simulink model "sonobe2025_explorer"  (R2025b)
settings: Solver=ode45  StartTime=0.0  StopTime=40  MaxStep=0.005  RelTol=1e-3
model workspace (MAT data in the model file):
  A = 62.8888888889
  Jb = 8
  Kd = 3.97
  Kp = 10.53
  Tv = 1
  g = 9.80665
  gamma = 0.02
  lb = 0.9
  mb = 60
  td = 0.155
settings Model: Creator=seguchi  LastModifiedBy=seguchi

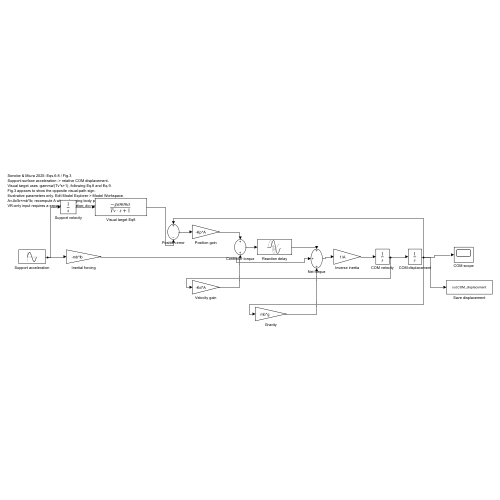
[thumbnail: Simulink's stored preview of the top-level diagram]
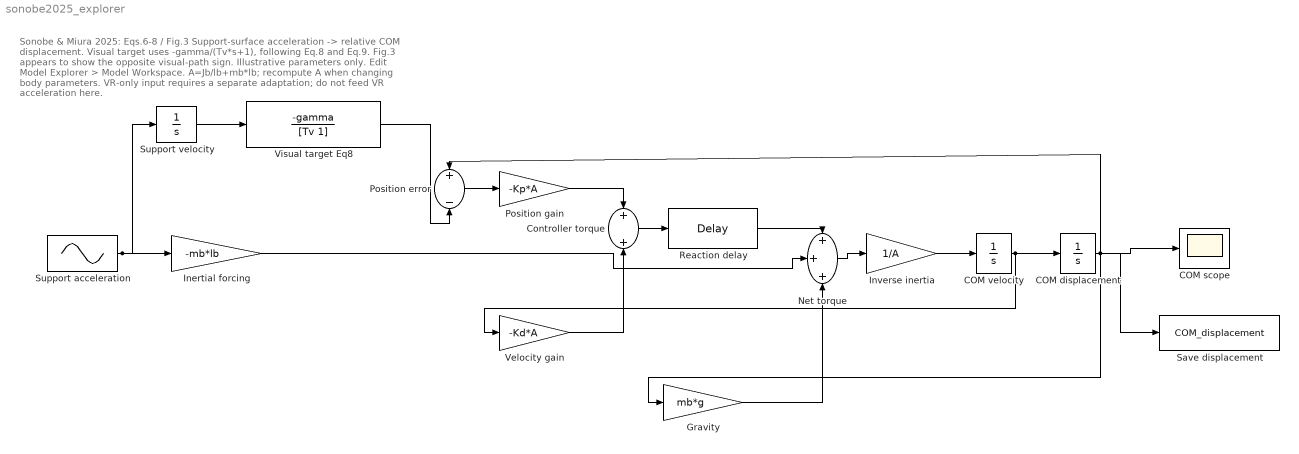
== system sonobe2025_explorer ==
  note: Sonobe & Miura 2025: Eqs.6-8 / Fig.3
      | Support-surface acceleration -> relative COM displacement.
      | Visual target uses -gamma/(Tv*s+1), following Eq.8 and Eq.9.
      | Fig.3 appears to show the opposite visual-path sign.
      | Illustrative parameters only. Edit Model Explorer > Model Workspace.
      | A=Jb/lb+mb*lb; recompute A when changing body parameters.
      | VR-only input requires a separate adaptation; do not feed VR acceleration here.
  COM displacement : Integrator
  COM scope : Scope
  COM velocity : Integrator
  Controller torque : Sum
  Gravity : Gain  Gain=mb*g
  Inertial forcing : Gain  Gain=-mb*lb
  Inverse inertia : Gain  Gain=1/A
  Net torque : Sum  Inputs=+++
  Position error : Sum  Inputs=+-
  Position gain : Gain  Gain=-Kp*A
  Reaction delay : TransportDelay  DelayTime=td
  Save displacement : ToWorkspace  VariableName=COM_displacement  SaveFormat=Timeseries  SampleTime=-1
  Support acceleration : Sin  Amplitude=0.02  Frequency=2*pi*0.2  SampleTime=0
  Support velocity : Integrator
  Velocity gain : Gain  Gain=-Kd*A
  Visual target Eq8 : TransferFcn  Numerator=-gamma  Denominator=[Tv 1]
  wires:
  Support acceleration/1 -> Support velocity/1, Inertial forcing/1
  Support velocity/1 -> Visual target Eq8/1
  Visual target Eq8/1 -> Position error/2
  COM displacement/1 -> Position error/1, Gravity/1, COM scope/1, Save displacement/1
  Position error/1 -> Position gain/1
  Position gain/1 -> Controller torque/1
  COM velocity/1 -> Velocity gain/1, COM displacement/1
  Velocity gain/1 -> Controller torque/2
  Controller torque/1 -> Reaction delay/1
  Reaction delay/1 -> Net torque/1
  Inertial forcing/1 -> Net torque/2
  Gravity/1 -> Net torque/3
  Net torque/1 -> Inverse inertia/1
  Inverse inertia/1 -> COM velocity/1
